simulink model "test3_ifelse"  (R2025b)
settings: Solver=ode45  StartTime=0.0  StopTime=100  MaxStep=0.01  RelTol=1e-3
settings Model: Creator=Shriram  LastModifiedBy=Shriram

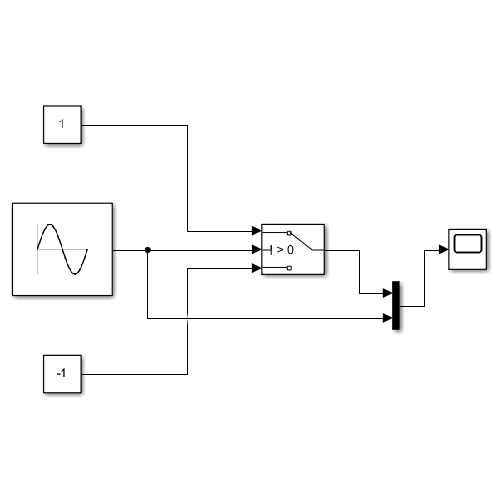
[thumbnail: Simulink's stored preview of the top-level diagram]
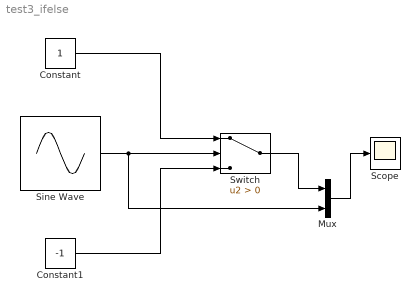
== system test3_ifelse ==
  Constant : Constant
  Constant1 : Constant  Value=-1
  Mux : Mux  Inputs=2
  Scope : Scope
      settings: ActiveDisplayYMinimum=-1.25  ActiveDisplayYMaximum=1.25
  Sine Wave : Sin  SampleTime=0
  Switch : Switch  Criteria=u2 > Threshold  SaturateOnIntegerOverflow=off  InputSameDT=off
  wires:
  Sine Wave/1 -> Mux/2, Switch/2
  Constant/1 -> Switch/1
  Constant1/1 -> Switch/3
  Switch/1 -> Mux/1
  Mux/1 -> Scope/1
